simulink model "phi5_m1_vr01_k5_2"  (R2026a)
settings: Solver=VariableStepAuto  StopTime=24.0
libraries: deeplib x1
settings Model: Creator=ldy  LastModifiedBy=harry_31916

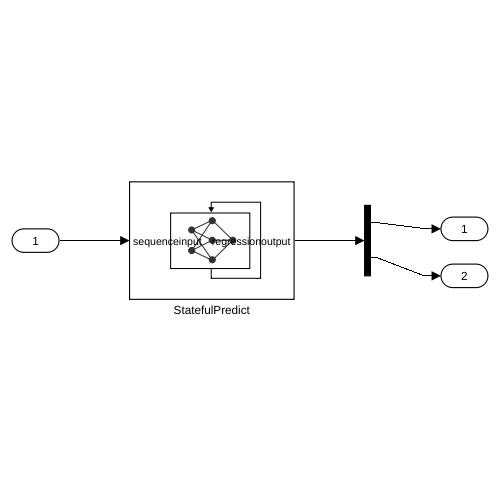
[thumbnail: Simulink's stored preview of the top-level diagram]
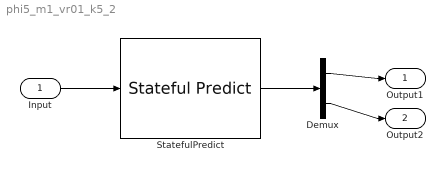
== system phi5_m1_vr01_k5_2 ==
  Input : Inport
  Demux : Demux  Outputs=2
  StatefulPredict : deeplib/Stateful Predict  Network=Network from MAT-file  NetworkFunction=untitled  NetworkFilePath=phi5_m1_vr01_k5_2.mat  SimulateUsing=Auto mode  InputDataFormats={'',''}  SampleTime=1  ForceInterpretedSim=off  EnableDLNetwork=on  LastKnownNetworkFilePath=''  LastKnownNetworkTimeStamp=''
  Output1 : Outport
  Output2 : Outport  Port=2
  wires:
  Input/1 -> StatefulPredict/1
  Demux/1 -> Output1/1
  Demux/2 -> Output2/1
  StatefulPredict/1 -> Demux/1
